simulink model "Trigger_FOC_Deadtime"  (R2022b)
settings: Solver=VariableStepAuto  StartTime=0.0  StopTime=0.5  RelTol=1e-3
PreLoadFcn:
  | % 沉沙motor:https://www.zhihu.com/people/gun-ne-ni
InitFcn:
  | %沉沙motor:https://www.zhihu.com/people/gun-ne-ni
  | 
  | deadtime = 2e-6;
undefined symbols (not defined in the file): Udc
libraries: spsGroundLib x1, spsPermanentMagnetSynchronousMachineLib x1, spsUniversalBridgeLib x1, spsDCVoltageSourceLib x1, sps_lib x1
settings Model: Creator=CSMotor  LastModifiedBy=CSMotor
settings DataIOCC: ReturnWorkspaceOutputs=off

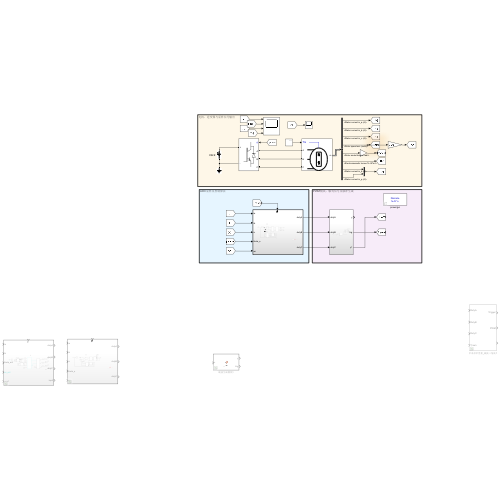
[thumbnail: Simulink's stored preview of the top-level diagram]
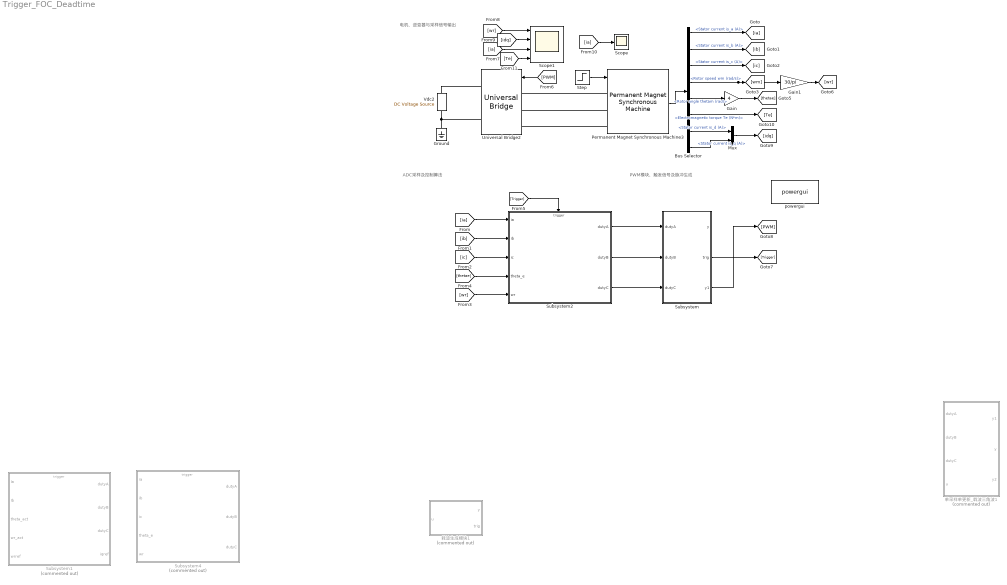
== system Trigger_FOC_Deadtime ==
  note: ADC采样及控制算法
  note: 电机、逆变器与采样信号输出
  note: PWM模块、触发信号及脉冲生成
  Bus Selector : BusSelector  OutputSignals=Stator current is_a (A),Stator current is_b (A),Stator current is_c (A),Rotor speed wm (rad/s),Rotor angle thetam (rad),Electromagnetic torque Te (N*m),Stator current is_d (A),Stator current is_q (A)
  Gain : Gain  Gain=4
  Gain1 : Gain  Gain=30/pi
  Ground : spsGroundLib/Ground  LConnTagsString=a
  Mux : Mux  Inputs=2
  Permanent Magnet Synchronous Machine3 : spsPermanentMagnetSynchronousMachineLib/Permanent Magnet Synchronous Machine  Description=沉沙motor:https://www.zhihu.com/people/gun-ne-ni  NbPhases=3  FluxDistribution=Sinusoidal  RotorType=Salient-pole  MechanicalLoad=Torque Tm  PresetModel="05:  8 Nm 300 Vdc 2000 RPM - 10 Nm"  ShowDetailedParameters=on  MeasurementBus=off  Resistance=0.9585  Inductance=8.5e-3  dqInductances=[0.004987 0.005513]  La=0.000835  MachineConstant=Flux linkage established by magnets (V.s)  Flux=0.1827  VoltageCst=132.5525  TorqueCst=1.0962  Flat=120  Mechanical=[0.0006329 0.0003035 4 0]  PolePairs=4  InitialConditions=[0,0, 0,0]  InitialConditions5ph=[0 0 0 0 0 0]  RefAngle=Aligned with phase A axis (original Park)  IterativeDiscreteModel=Trapezoidal non iterative  TsBlock=-1  TsPowergui=0
  Scope : Scope
  Scope1 : Scope  NumInputPorts=4
  Step : Step  Time=0.25  After=5  SampleTime=0
  Subsystem : Subsystem
  Subsystem1 : Subsystem  Commented=on
  Subsystem2 : Subsystem
  Subsystem4 : Subsystem  Commented=on
  Universal Bridge2 : spsUniversalBridgeLib/Universal Bridge  Description=沉沙motor:https://www.zhihu.com/people/gun-ne-ni  Arms=3  SnubberResistance=1e5  SnubberCapacitance=inf  Device=IGBT / Diodes  Ron=1e-3  Lon=0  ForwardVoltages="[  0  0  ]"  ForwardVoltage=0  GTOparameters=[ 10e-6 , 20e-6 ]  IGBTparameters=[ 1e-6 , 2e-6 ]  Measurements=None  Measurements_2=None  converterType=Rectifier
  Vdc2 : spsDCVoltageSourceLib/DC Voltage Source  Amplitude=300  Measurements=None
  powergui : sps_lib/powergui  Priority=1  SimulationMode=Discrete  SampleTime=1e-7  frequency=60  Iterations=50  frequencyindice=0  Pbase=100e6  ErrMax=1e-4  UnitsV=kV  UnitsW=MW  buscounter=0  FunctionMessages=off  echomessages=off  EnableUseOfTLC=off  CurrentSourceSwitches=off  DisableSnubberDevices=off  DisableRonSwitches=off  DisableVfSwitches=off  DisplayEquations=off  AutomaticDiscreteSolvers=off  SolverType=Tustin/Backward Euler (TBE)  Interpol=off  ExternalGateDelay=off  methode=off  Ts=100  x0status=blocks  SPID=on  SwTol=0  HookPort=off  NonlinearTolerance=1e-4  nMaxIteration=100  ContinueOnMaxIteration=off  RestoreLinks=warning  ResistiveCurrentMeasurement=off  Frange=[0:2:500]  Ylog=off  Xlog=on  ShowGrid=off  save=off  variable=ZData  structure=0  ZoomFFT=off  StartTime=0.0  cycles=1  DisplayStyle=1  fundamental=60  FreqAxis=off  MaxFrequency=1000  frequencyindicesteady=1  RmsSteady=1  display=off
  单采样单更新_载波三角波1 : Subsystem  Commented=on
      mask Display:
      | port_label('output',1,'Trigger')
      | port_label('output',2,'PWM')
      | 
      | 
      | 
      | port_label('input',1,'DutyA')
      | port_label('input',2,'DutyB')
      | port_label('input',3,'DutyC')
      | port_label('input',4,'Tpwm')
  载波生成模块1 : MATLAB Function  Commented=on  TreatAsAtomicUnit=on
  wires:
  Permanent Magnet Synchronous Machine3/1 -> Bus Selector/1
  Bus Selector/1 -> [ia]  "<Stator current is_a (A)>"
  Bus Selector/2 -> [ib]  "<Stator current is_b (A)>"
  Bus Selector/3 -> [ic]  "<Stator current is_c (A)>"
  Bus Selector/4 -> Gain1/1, [wm]  "<Rotor speed wm (rad/s)>"
  Bus Selector/5 -> Gain/1  "<Rotor angle thetam (rad)>"
  Gain/1 -> [thetae]
  Gain1/1 -> [wr]
  [PWM] -> Universal Bridge2/1
  [wr] -> Subsystem2/5(wr)
  [Trigger] -> Subsystem2/Trigger
  [ia] -> Subsystem2/1(ia)
  [ib] -> Subsystem2/2(ib)
  [ic] -> Subsystem2/3(ic)
  [thetae] -> Subsystem2/4(theta_e)
  Subsystem/2(trig) -> [Trigger]
  Subsystem2/1(dutyA) -> Subsystem/1(dutyA)
  Subsystem2/2(dutyB) -> Subsystem/2(dutyB)
  Subsystem2/3(dutyC) -> Subsystem/3(dutyC)
  Step/1 -> Permanent Magnet Synchronous Machine3/1
  [wr] -> Scope1/1
  [ia] -> Scope1/3
  Bus Selector/7 -> Mux/1  "<Stator current is_d (A)>"
  Bus Selector/8 -> Mux/2  "<Stator current is_q (A)>"
  Mux/1 -> [idq]
  [idq] -> Scope1/2
  Bus Selector/6 -> [Te]  "<Electromagnetic torque Te (N*m)>"
  [Te] -> Scope1/4
  [ia] -> Scope/1
  Subsystem/3(y1) -> [PWM]
  connections:
  Permanent Magnet Synchronous Machine3/LConn1 -- Universal Bridge2/LConn1
  Permanent Magnet Synchronous Machine3/LConn2 -- Universal Bridge2/LConn2
  Permanent Magnet Synchronous Machine3/LConn3 -- Universal Bridge2/LConn3
  Vdc2/RConn1 -- Universal Bridge2/RConn1
  Vdc2/LConn1 -- Ground/LConn1 -- Universal Bridge2/RConn2

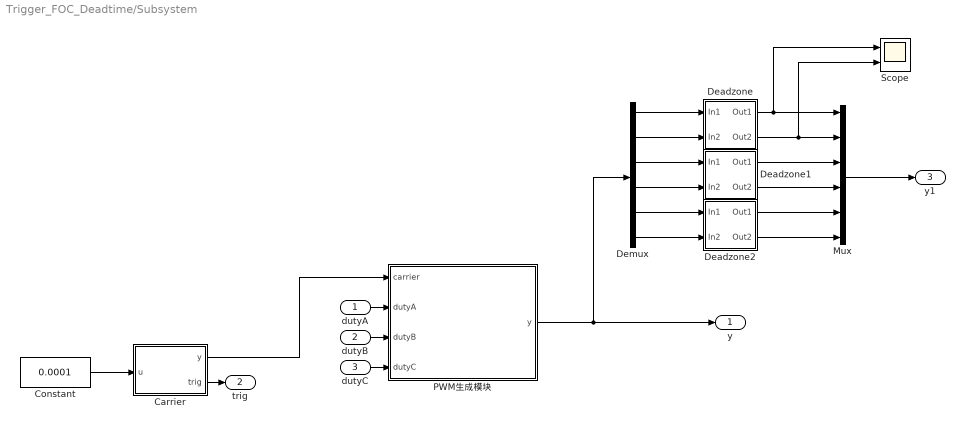
== system Trigger_FOC_Deadtime/Subsystem ==
  dutyA : Inport
  dutyB : Inport  Port=2
  dutyC : Inport  Port=3
  Carrier : MATLAB Function  Description=沉沙motor:https://www.zhihu.com/people/gun-ne-ni  TreatAsAtomicUnit=on
  Constant : Constant  Value=0.0001
  Deadzone : Subsystem
  Deadzone1 : Subsystem
  Deadzone2 : Subsystem
  Demux : Demux  Outputs=6
  Mux : Mux  Inputs=6
  PWM生成模块 : MATLAB Function  Description=沉沙motor:https://www.zhihu.com/people/gun-ne-ni  TreatAsAtomicUnit=on
  Scope : Scope  NumInputPorts=2
  y : Outport
  trig : Outport  Port=2
  y1 : Outport  Port=3
  wires:
  Carrier/1(y) -> PWM生成模块/1(carrier)
  PWM生成模块/1(y) -> Demux/1, y/1
  dutyC/1 -> PWM生成模块/4(dutyC)
  Constant/1 -> Carrier/1(u)
  dutyA/1 -> PWM生成模块/2(dutyA)
  dutyB/1 -> PWM生成模块/3(dutyB)
  Carrier/2(trig) -> trig/1
  Demux/1 -> Deadzone/1(In1)
  Demux/2 -> Deadzone/2(In2)
  Deadzone/2(Out2) -> Scope/2, Mux/2
  Deadzone/1(Out1) -> Scope/1, Mux/1
  Demux/3 -> Deadzone1/1(In1)
  Demux/4 -> Deadzone1/2(In2)
  Deadzone1/1(Out1) -> Mux/3
  Deadzone1/2(Out2) -> Mux/4
  Demux/5 -> Deadzone2/1(In1)
  Demux/6 -> Deadzone2/2(In2)
  Deadzone2/1(Out1) -> Mux/5
  Deadzone2/2(Out2) -> Mux/6
  Mux/1 -> y1/1

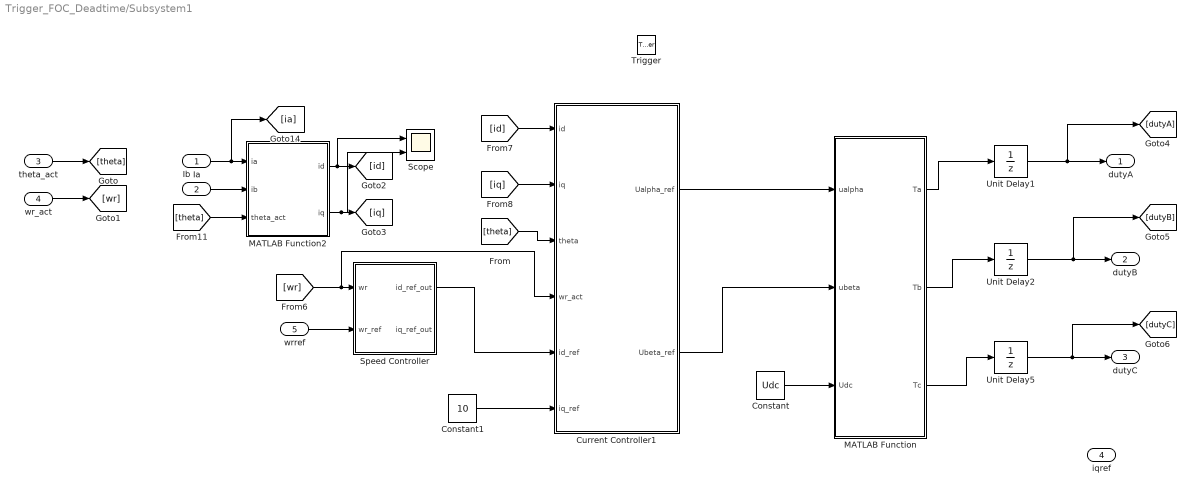
== system Trigger_FOC_Deadtime/Subsystem1 ==
  Ia : Inport
  Ib : Inport  Port=2
  theta_act : Inport  Port=3
  wr_act : Inport  Port=4
  wrref : Inport  Port=5
  Trigger : TriggerPort  VariantControl=(inherit)  PortDimensions=1
  Constant : Constant  Value=Udc
  Constant1 : Constant  Value=10
  Current Controller1 : MATLAB Function  TreatAsAtomicUnit=on
  MATLAB Function : MATLAB Function  TreatAsAtomicUnit=on
  MATLAB Function2 : MATLAB Function  TreatAsAtomicUnit=on
  Scope : Scope  NumInputPorts=2
  Speed Controller : MATLAB Function  TreatAsAtomicUnit=on
  Unit Delay1 : UnitDelay  InitialCondition=1e-4  SampleTime=-1  HasFrameUpgradeWarning=on
  Unit Delay2 : UnitDelay  InitialCondition=1e-4  SampleTime=-1  HasFrameUpgradeWarning=on
  Unit Delay5 : UnitDelay  InitialCondition=1e-4  SampleTime=-1  HasFrameUpgradeWarning=on
  dutyA : Outport
  dutyB : Outport  Port=2
  dutyC : Outport  Port=3
  iqref : Outport  Port=4
  wires:
  Constant1/1 -> Current Controller1/6(iq_ref)
  [iq] -> Current Controller1/2(iq)
  MATLAB Function2/1(id) -> [id], Scope/1
  MATLAB Function/2(Tb) -> Unit Delay2/1
  [id] -> Current Controller1/1(id)
  Unit Delay5/1 -> [dutyC], dutyC/1
  MATLAB Function/3(Tc) -> Unit Delay5/1
  Unit Delay1/1 -> [dutyA], dutyA/1
  Current Controller1/2(Ubeta_ref) -> MATLAB Function/2(ubeta)
  MATLAB Function/1(Ta) -> Unit Delay1/1
  MATLAB Function2/2(iq) -> [iq], Scope/2
  Ib/1 -> MATLAB Function2/2(ib)
  wrref/1 -> Speed Controller/2(wr_ref)
  Ia/1 -> [ia], MATLAB Function2/1(ia)
  [theta] -> MATLAB Function2/3(theta_act)
  [wr] -> Current Controller1/4(wr_act), Speed Controller/1(wr)
  Unit Delay2/1 -> [dutyB], dutyB/1
  [theta] -> Current Controller1/3(theta)
  Constant/1 -> MATLAB Function/3(Udc)
  Current Controller1/1(Ualpha_ref) -> MATLAB Function/1(ualpha)
  theta_act/1 -> [theta]
  Speed Controller/1(id_ref_out) -> Current Controller1/5(id_ref)
  wr_act/1 -> [wr]

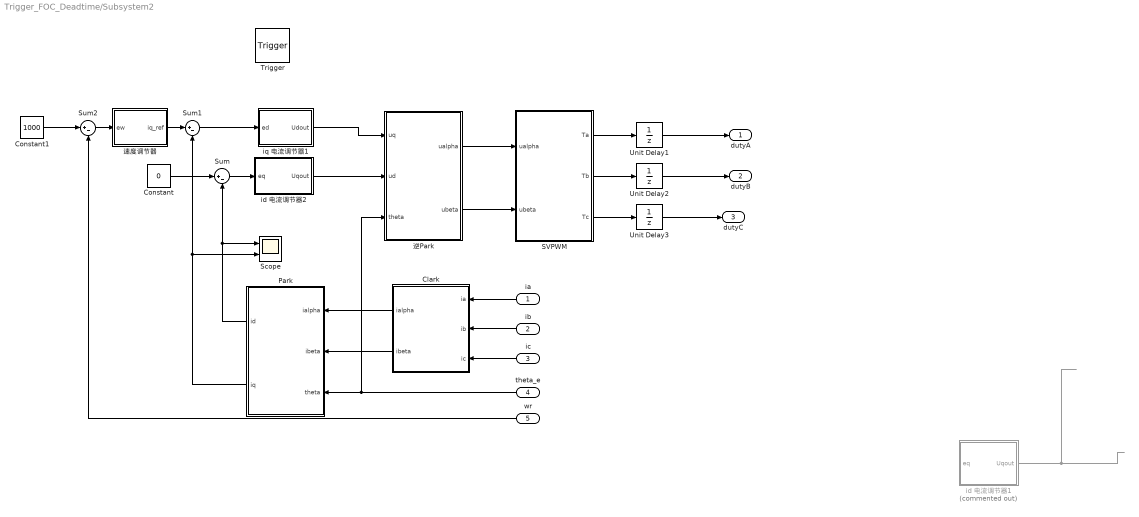
== system Trigger_FOC_Deadtime/Subsystem2 ==
  ia : Inport
  ib : Inport  Port=2
  ic : Inport  Port=3
  theta_e : Inport  Port=4
  wr : Inport  Port=5
  Trigger : TriggerPort  VariantControl=(inherit)  PortDimensions=1
  Clark : MATLAB Function  Description=沉沙motor:https://www.zhihu.com/people/gun-ne-ni  TreatAsAtomicUnit=on
  Constant : Constant  Value=0
  Constant1 : Constant  Value=1000
  Park : MATLAB Function  Description=沉沙motor:https://www.zhihu.com/people/gun-ne-ni  TreatAsAtomicUnit=on
  SVPWM : MATLAB Function  Description=沉沙motor:https://www.zhihu.com/people/gun-ne-ni  TreatAsAtomicUnit=on
  Scope : Scope  NumInputPorts=2
  Sum : Sum  Inputs=|+-
  Sum1 : Sum  Inputs=|+-
  Sum2 : Sum  Inputs=|+-
  Unit Delay1 : UnitDelay  InitialCondition=1e-4  SampleTime=-1  HasFrameUpgradeWarning=on
  Unit Delay2 : UnitDelay  InitialCondition=1e-4  SampleTime=-1  HasFrameUpgradeWarning=on
  Unit Delay3 : UnitDelay  InitialCondition=1e-4  SampleTime=-1  HasFrameUpgradeWarning=on
  id 电流调节器1 : MATLAB Function  Commented=on  TreatAsAtomicUnit=on
  id 电流调节器2 : MATLAB Function  Tag=s  Description=沉沙motor:https://www.zhihu.com/people/gun-ne-ni  TreatAsAtomicUnit=on
  iq 电流调节器1 : MATLAB Function  Description=沉沙motor:https://www.zhihu.com/people/gun-ne-ni  TreatAsAtomicUnit=on
  逆Park : MATLAB Function  Description=沉沙motor:https://www.zhihu.com/people/gun-ne-ni  TreatAsAtomicUnit=on
  速度调节器 : MATLAB Function  TreatAsAtomicUnit=on
  dutyA : Outport
  dutyB : Outport  Port=2
  dutyC : Outport  Port=3
  wires:
  id 电流调节器1/1(Uqout) -> ?
  SVPWM/3(Tc) -> Unit Delay3/1
  SVPWM/2(Tb) -> Unit Delay2/1
  SVPWM/1(Ta) -> Unit Delay1/1
  Constant1/1 -> Sum2/1
  wr/1 -> Sum2/2
  Sum2/1 -> 速度调节器/1(ew)
  Park/2(iq) -> Scope/2, Sum1/2
  Clark/2(ibeta) -> Park/2(ibeta)
  Clark/1(ialpha) -> Park/1(ialpha)
  theta_e/1 -> Park/3(theta), 逆Park/3(theta)
  ic/1 -> Clark/3(ic)
  ib/1 -> Clark/2(ib)
  ia/1 -> Clark/1(ia)
  逆Park/1(ualpha) -> SVPWM/1(ualpha)
  逆Park/2(ubeta) -> SVPWM/2(ubeta)
  Sum/1 -> id 电流调节器2/1(eq)
  Constant/1 -> Sum/1
  速度调节器/1(iq_ref) -> Sum1/1
  Sum1/1 -> iq 电流调节器1/1(ed)
  iq 电流调节器1/1(Udout) -> 逆Park/1(uq)
  id 电流调节器2/1(Uqout) -> 逆Park/2(ud)
  Park/1(id) -> Sum/2, Scope/1
  Unit Delay1/1 -> dutyA/1
  Unit Delay2/1 -> dutyB/1
  Unit Delay3/1 -> dutyC/1

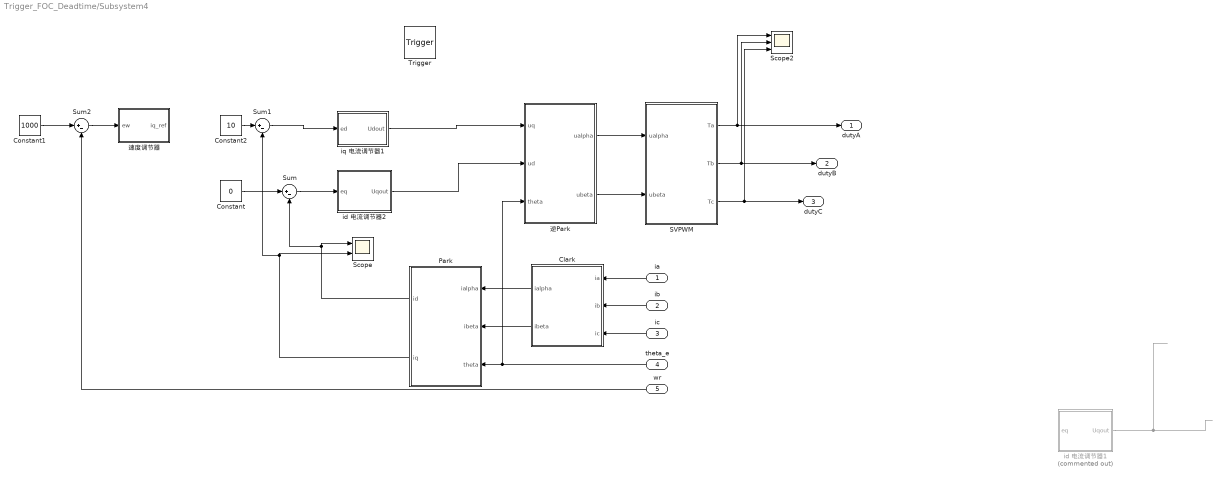
== system Trigger_FOC_Deadtime/Subsystem4 ==
  ia : Inport
  ib : Inport  Port=2
  ic : Inport  Port=3
  theta_e : Inport  Port=4
  wr : Inport  Port=5
  Trigger : TriggerPort  VariantControl=(inherit)  PortDimensions=1
  Clark : MATLAB Function  TreatAsAtomicUnit=on
  Constant : Constant  Value=0
  Constant1 : Constant  Value=1000
  Constant2 : Constant  Value=10
  Park : MATLAB Function  TreatAsAtomicUnit=on
  SVPWM : MATLAB Function  TreatAsAtomicUnit=on
  Scope : Scope  NumInputPorts=2
  Scope2 : Scope  NumInputPorts=3
  Sum : Sum  Inputs=|+-
  Sum1 : Sum  Inputs=|+-
  Sum2 : Sum  Inputs=|+-
  id 电流调节器1 : MATLAB Function  Commented=on  TreatAsAtomicUnit=on
  id 电流调节器2 : MATLAB Function  TreatAsAtomicUnit=on
  iq 电流调节器1 : MATLAB Function  TreatAsAtomicUnit=on
  逆Park : MATLAB Function  TreatAsAtomicUnit=on
  速度调节器 : MATLAB Function  TreatAsAtomicUnit=on
  dutyA : Outport
  dutyB : Outport  Port=2
  dutyC : Outport  Port=3
  wires:
  id 电流调节器2/1(Uqout) -> 逆Park/2(ud)
  iq 电流调节器1/1(Udout) -> 逆Park/1(uq)
  Sum1/1 -> iq 电流调节器1/1(ed)
  Constant2/1 -> Sum1/1
  Park/1(id) -> Scope/1, Sum/2
  Constant/1 -> Sum/1
  Sum/1 -> id 电流调节器2/1(eq)
  逆Park/2(ubeta) -> SVPWM/2(ubeta)
  逆Park/1(ualpha) -> SVPWM/1(ualpha)
  ia/1 -> Clark/1(ia)
  ib/1 -> Clark/2(ib)
  ic/1 -> Clark/3(ic)
  theta_e/1 -> 逆Park/3(theta), Park/3(theta)
  Clark/1(ialpha) -> Park/1(ialpha)
  Clark/2(ibeta) -> Park/2(ibeta)
  Park/2(iq) -> Scope/2, Sum1/2
  Sum2/1 -> 速度调节器/1(ew)
  wr/1 -> Sum2/2
  Constant1/1 -> Sum2/1
  SVPWM/1(Ta) -> Scope2/1, dutyA/1
  SVPWM/2(Tb) -> Scope2/2, dutyB/1
  SVPWM/3(Tc) -> Scope2/3, dutyC/1
  id 电流调节器1/1(Uqout) -> ?

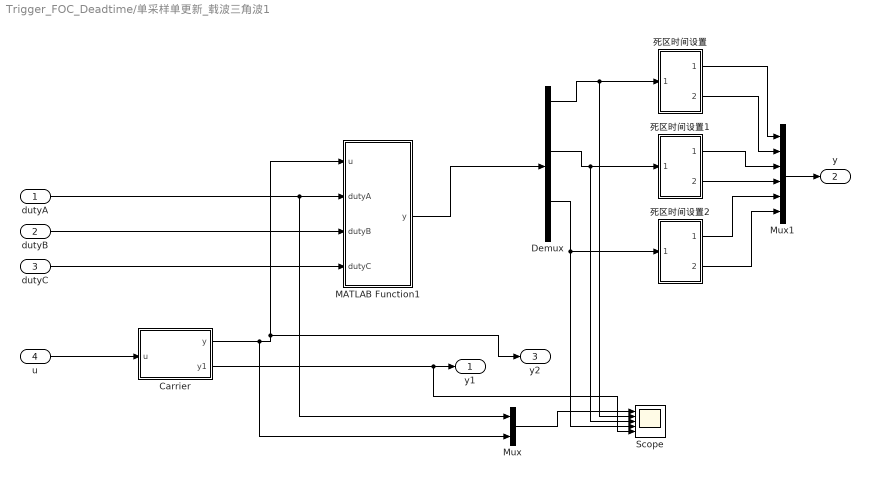
== system Trigger_FOC_Deadtime/单采样单更新_载波三角波1 ==
  dutyA : Inport
  dutyB : Inport  Port=2
  dutyC : Inport  Port=3
  u : Inport  Port=4
  Carrier : MATLAB Function  TreatAsAtomicUnit=on
  Demux : Demux  Outputs=6
  MATLAB Function1 : MATLAB Function  TreatAsAtomicUnit=on
  Mux : Mux  Inputs=2
  Mux1 : Mux  Inputs=6
  Scope : Scope  NumInputPorts=5
  死区时间设置 : Subsystem
  死区时间设置1 : Subsystem
  死区时间设置2 : Subsystem
  y1 : Outport
  y : Outport  Port=2
  y2 : Outport  Port=3
  wires:
  Carrier/2(y1) -> y1/1, Scope/5
  死区时间设置2/2(Out2) -> Mux1/6
  死区时间设置2/1(Out1) -> Mux1/5
  死区时间设置1/2(Out2) -> Mux1/4
  死区时间设置1/1(Out1) -> Mux1/3
  死区时间设置/2(Out2) -> Mux1/2
  死区时间设置/1(Out1) -> Mux1/1
  Demux/5 -> Scope/4, 死区时间设置2/1(In1)
  Demux/3 -> Scope/3, 死区时间设置1/1(In1)
  dutyA/1 -> Mux/1, MATLAB Function1/2(dutyA)
  MATLAB Function1/1(y) -> Demux/1
  u/1 -> Carrier/1(u)
  Carrier/1(y) -> Mux/2, y2/1, MATLAB Function1/1(u)
  dutyB/1 -> MATLAB Function1/3(dutyB)
  dutyC/1 -> MATLAB Function1/4(dutyC)
  Demux/1 -> Scope/2, 死区时间设置/1(In1)
  Mux/1 -> Scope/1
  Mux1/1 -> y/1

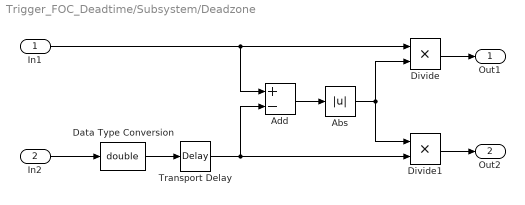
== system Trigger_FOC_Deadtime/Subsystem/Deadzone ==
  In1 : Inport
  In2 : Inport  Port=2
  Abs : Abs  SaturateOnIntegerOverflow=off
  Add : Sum  Inputs=+-
  Data Type Conversion : DataTypeConversion  OutDataTypeStr=double  SaturateOnIntegerOverflow=off  RndMeth=Floor
  Divide : Product  Inputs=**
  Divide1 : Product  Inputs=**
  Transport Delay : TransportDelay  DelayTime=2e-6
  Out1 : Outport  VectorParamsAs1DForOutWhenUnconnected=off
  Out2 : Outport  Port=2  VectorParamsAs1DForOutWhenUnconnected=off
  wires:
  Abs/1 -> Divide1/1, Divide/2
  Data Type Conversion/1 -> Transport Delay/1
  Add/1 -> Abs/1
  Transport Delay/1 -> Add/2, Divide1/2
  Divide/1 -> Out1/1
  In2/1 -> Data Type Conversion/1
  In1/1 -> Divide/1, Add/1
  Divide1/1 -> Out2/1

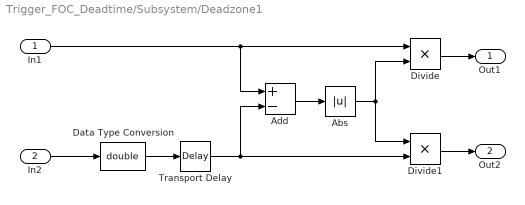
== system Trigger_FOC_Deadtime/Subsystem/Deadzone1 ==
  In1 : Inport
  In2 : Inport  Port=2
  Abs : Abs  SaturateOnIntegerOverflow=off
  Add : Sum  Inputs=+-
  Data Type Conversion : DataTypeConversion  OutDataTypeStr=double  SaturateOnIntegerOverflow=off  RndMeth=Floor
  Divide : Product  Inputs=**
  Divide1 : Product  Inputs=**
  Transport Delay : TransportDelay  DelayTime=2e-6
  Out1 : Outport  VectorParamsAs1DForOutWhenUnconnected=off
  Out2 : Outport  Port=2  VectorParamsAs1DForOutWhenUnconnected=off
  wires:
  Divide1/1 -> Out2/1
  In1/1 -> Add/1, Divide/1
  In2/1 -> Data Type Conversion/1
  Divide/1 -> Out1/1
  Transport Delay/1 -> Divide1/2, Add/2
  Add/1 -> Abs/1
  Data Type Conversion/1 -> Transport Delay/1
  Abs/1 -> Divide/2, Divide1/1

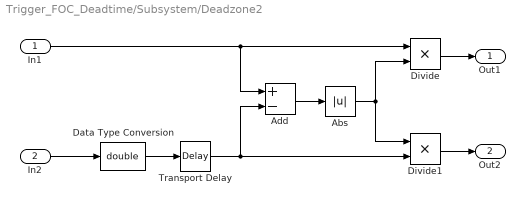
== system Trigger_FOC_Deadtime/Subsystem/Deadzone2 ==
  In1 : Inport
  In2 : Inport  Port=2
  Abs : Abs  SaturateOnIntegerOverflow=off
  Add : Sum  Inputs=+-
  Data Type Conversion : DataTypeConversion  OutDataTypeStr=double  SaturateOnIntegerOverflow=off  RndMeth=Floor
  Divide : Product  Inputs=**
  Divide1 : Product  Inputs=**
  Transport Delay : TransportDelay  DelayTime=2e-6
  Out1 : Outport  VectorParamsAs1DForOutWhenUnconnected=off
  Out2 : Outport  Port=2  VectorParamsAs1DForOutWhenUnconnected=off
  wires:
  Abs/1 -> Divide1/1, Divide/2
  Data Type Conversion/1 -> Transport Delay/1
  Add/1 -> Abs/1
  Transport Delay/1 -> Add/2, Divide1/2
  Divide/1 -> Out1/1
  In2/1 -> Data Type Conversion/1
  In1/1 -> Divide/1, Add/1
  Divide1/1 -> Out2/1

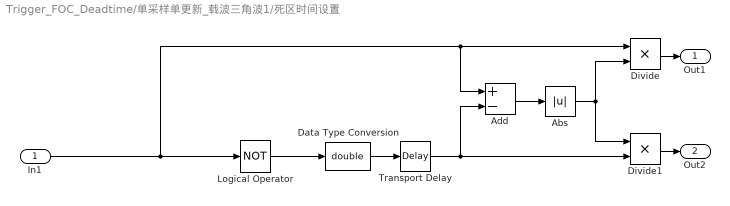
== system Trigger_FOC_Deadtime/单采样单更新_载波三角波1/死区时间设置 ==
  In1 : Inport
  Abs : Abs  SaturateOnIntegerOverflow=off
  Add : Sum  Inputs=+-
  Data Type Conversion : DataTypeConversion  OutDataTypeStr=double  SaturateOnIntegerOverflow=off  RndMeth=Floor
  Divide : Product  Inputs=**
  Divide1 : Product  Inputs=**
  Logical Operator : Logic  Operator=NOT  AllPortsSameDT=off  OutDataTypeStr=boolean
  Transport Delay : TransportDelay  DelayTime=deadtime
  Out1 : Outport  VectorParamsAs1DForOutWhenUnconnected=off
  Out2 : Outport  Port=2  VectorParamsAs1DForOutWhenUnconnected=off
  wires:
  Add/1 -> Abs/1
  Divide1/1 -> Out2/1
  Logical Operator/1 -> Data Type Conversion/1
  Divide/1 -> Out1/1
  Abs/1 -> Divide/2, Divide1/1
  In1/1 -> Add/1, Divide/1, Logical Operator/1
  Transport Delay/1 -> Divide1/2, Add/2
  Data Type Conversion/1 -> Transport Delay/1

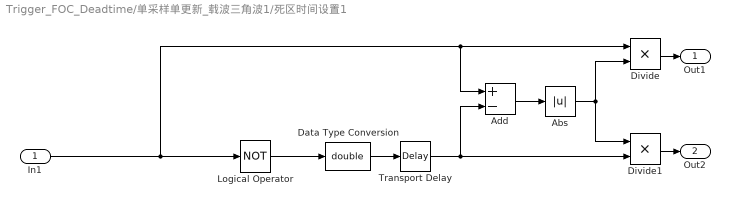
== system Trigger_FOC_Deadtime/单采样单更新_载波三角波1/死区时间设置1 ==
  In1 : Inport
  Abs : Abs  SaturateOnIntegerOverflow=off
  Add : Sum  Inputs=+-
  Data Type Conversion : DataTypeConversion  OutDataTypeStr=double  SaturateOnIntegerOverflow=off  RndMeth=Floor
  Divide : Product  Inputs=**
  Divide1 : Product  Inputs=**
  Logical Operator : Logic  Operator=NOT  AllPortsSameDT=off  OutDataTypeStr=boolean
  Transport Delay : TransportDelay  DelayTime=deadtime
  Out1 : Outport  VectorParamsAs1DForOutWhenUnconnected=off
  Out2 : Outport  Port=2  VectorParamsAs1DForOutWhenUnconnected=off
  wires:
  Data Type Conversion/1 -> Transport Delay/1
  Transport Delay/1 -> Add/2, Divide1/2
  In1/1 -> Logical Operator/1, Divide/1, Add/1
  Abs/1 -> Divide1/1, Divide/2
  Divide/1 -> Out1/1
  Logical Operator/1 -> Data Type Conversion/1
  Divide1/1 -> Out2/1
  Add/1 -> Abs/1

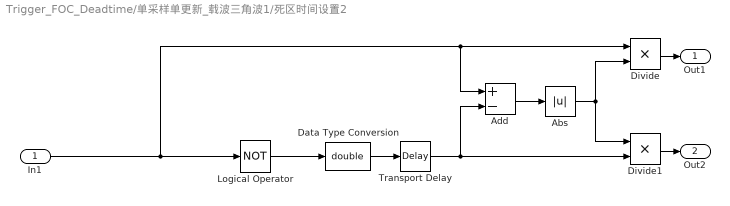
== system Trigger_FOC_Deadtime/单采样单更新_载波三角波1/死区时间设置2 ==
  In1 : Inport
  Abs : Abs  SaturateOnIntegerOverflow=off
  Add : Sum  Inputs=+-
  Data Type Conversion : DataTypeConversion  OutDataTypeStr=double  SaturateOnIntegerOverflow=off  RndMeth=Floor
  Divide : Product  Inputs=**
  Divide1 : Product  Inputs=**
  Logical Operator : Logic  Operator=NOT  AllPortsSameDT=off  OutDataTypeStr=boolean
  Transport Delay : TransportDelay  DelayTime=deadtime
  Out1 : Outport  VectorParamsAs1DForOutWhenUnconnected=off
  Out2 : Outport  Port=2  VectorParamsAs1DForOutWhenUnconnected=off
  wires:
  Add/1 -> Abs/1
  Divide1/1 -> Out2/1
  Logical Operator/1 -> Data Type Conversion/1
  Divide/1 -> Out1/1
  Abs/1 -> Divide/2, Divide1/1
  In1/1 -> Add/1, Divide/1, Logical Operator/1
  Transport Delay/1 -> Divide1/2, Add/2
  Data Type Conversion/1 -> Transport Delay/1

== matlab function Trigger_FOC_Deadtime/Subsystem4/Park ==
  data: ialpha input; id output; ibeta input; theta input; iq output
function [id, iq] = fcn(ialpha, ibeta, theta)
%#codegen
id =  ialpha*cos(theta) + ibeta*sin(theta);
iq = -ialpha*sin(theta) + ibeta*cos(theta);

== matlab function Trigger_FOC_Deadtime/Subsystem2/Clark ==
  data: ia input; ialpha output; ib input; ic input; ibeta output
function [ialpha, ibeta] = fcn_clarke(ia, ib, ic)
%#codegen
ialpha = (2/3) * (ia - 0.5*ib - 0.5*ic);
ibeta  = (2/3) * (sqrt(3)/2*ib - sqrt(3)/2*ic);

== matlab function Trigger_FOC_Deadtime/Subsystem/PWM生成模块 ==
  data: carrier input; y output; dutyA input; dutyB input; dutyC input
function y = fcn(carrier, dutyA, dutyB, dutyC)
%#codegen
ref  = carrier;
CMPA = dutyA;
CMPB = dutyB;
CMPC = dutyC;

Ta1 = 0;  Ta2 = 0;
Tb1 = 0;  Tb2 = 0;
Tc1 = 0;  Tc2 = 0;

if ref <= CMPA
    Ta1 = 1;  Ta2 = 0;
else
    Ta1 = 0;  Ta2 = 1;
end

if ref <= CMPB
    Tb1 = 1;  Tb2 = 0;
else
    Tb1 = 0;  Tb2 = 1;
end

if ref <= CMPC
    Tc1 = 1;  Tc2 = 0;
else
    Tc1 = 0;  Tc2 = 1;
end

y = [Ta1; Ta2; Tb1; Tb2; Tc1; Tc2];

== matlab function Trigger_FOC_Deadtime/Subsystem/Carrier ==
  data: u input; y output; trig output
function [y, trig] = carrier(u)
%#codegen
persistent cnt dir
if isempty(cnt)
    cnt = 0;
    dir = 1;
end
Tdis = 1e-7;
n  = round(u/Tdis);
nh = n/2;

y = cnt/nh;
trig = (cnt == nh);

cnt = cnt + dir;
if cnt >= nh
    cnt = nh;
    dir = -1;
elseif cnt <= 0
    cnt = 0;
    dir = 1;
end

== matlab function Trigger_FOC_Deadtime/载波生成模块1 ==
  data: u input; y output; trig output
function [y, trig] = carrier(u)
%#codegen
persistent cnt dir
if isempty(cnt)
    cnt = 0;
    dir = 1;
end
Tdis = 1e-7;
n  = round(u/Tdis);
nh = n/2;

y = cnt/nh;
trig = (cnt == nh);

cnt = cnt + dir;
if cnt >= nh
    cnt = nh;
    dir = -1;
elseif cnt <= 0
    cnt = 0;
    dir = 1;
end

== matlab function Trigger_FOC_Deadtime/Subsystem1/Current Controller1 ==
  data: id input; iq input; theta input; wr_act input; id_ref input; iq_ref input; Ualpha_ref output; Ubeta_ref output
function [Ualpha_ref,Ubeta_ref]  = fcn(id, iq, theta, wr_act, id_ref, iq_ref)
    persistent int_d int_q Kp Ki Ld Lq Phif Pn Tsc U_max Rs
    if isempty(int_d)
        int_d = 0;
        int_q = 0;
        Ld = 0.08e-3;
        Lq = 0.08e-3;
        Rs = 0.06;
        Phif = 0.003749;
        Pn = 5;
        Tsc = 0.0001;
        U_max = 24/sqrt(3);
    end
    
        Kp = Ld/4/Tsc;
        Ki = Rs/3/Tsc;

    we = wr_act * (2*pi/60) * Pn;
    
    err_d = id_ref - id;
    err_q = iq_ref - iq;
    
    int_d = int_d + Ki * err_d * Tsc;
    int_q = int_q + Ki * err_q * Tsc;

    %%%%%%%%% 积分限幅 %%%%%%%%%%%%
    if int_d > U_max 
        int_d = U_max;
    elseif int_d < -U_max
        int_d = -U_max;
    else
    end

    if int_q > U_max 
        int_q = U_max;
    elseif int_q < -U_max
        int_q = -U_max;
    else
    end

    %%%%%%%%%%% PI 输出 %%%%%%%%%%%
    Ud_raw = Kp * err_d + int_d;
    Uq_raw = Kp * err_q + int_q;
    
    
    U_mag = sqrt(Ud_raw^2 + Uq_raw^2);
    if U_mag > U_max
        scale = U_max / U_mag;
        Udout = Ud_raw * scale;
        Uqout = Uq_raw * scale;
    else
        Udout = Ud_raw;
        Uqout = Uq_raw;
    end
    
    theta_comp = theta + 1.5 * we * Tsc;
    Ualpha_ref = Udout * cos(theta_comp) - Uqout * sin(theta_comp);
    Ubeta_ref  = Udout * sin(theta_comp) + Uqout * cos(theta_comp);
end

== matlab function Trigger_FOC_Deadtime/Subsystem4/SVPWM ==
  data: ualpha input; Ta output; ubeta input; Tb output; Tc output
function [Ta, Tb, Tc] = fcn_svpwm(ualpha, ubeta)
%#codegen
SQRT3     = 1.73205080757;
SQRT3_INV = 0.57735026919;
Udc  = 300;

volAlphaNorm = ualpha/Udc*SQRT3;
volBetaNorm  = ubeta /Udc*SQRT3;

voltU = volAlphaNorm;
voltV = -0.5*volAlphaNorm + SQRT3*0.5*volBetaNorm;
voltW = -0.5*volAlphaNorm - SQRT3*0.5*volBetaNorm;

voltMax = max([voltU, voltV, voltW]);
voltMin = min([voltU, voltV, voltW]);
voltZero = -0.5*(voltMax + voltMin);

dutyU = SQRT3_INV*(voltU + voltZero) + 0.5;
dutyV = SQRT3_INV*(voltV + voltZero) + 0.5;
dutyW = SQRT3_INV*(voltW + voltZero) + 0.5;

Ta = min(max(dutyU, 0), 1);
Tb = min(max(dutyV, 0), 1);
Tc = min(max(dutyW, 0), 1);

== matlab function Trigger_FOC_Deadtime/Subsystem4/id 电流调节器1 ==
  data: eq input; Uqout output
function Uqout = fcn_pi_q(eq)
%#codegen
Lq  = 0.005513;
Rs  = 0.9585;
Tsc = 0.0001;
Udc = 300;

Kpq = Lq/(3*Tsc);
Kiq = Rs/(3*Tsc);
Umax = max(Udc,0)/sqrt(3);

persistent int_q
if isempty(int_q)
    int_q = 0;
end

int_q = int_q + Kiq*eq*Tsc;

if int_q >  Umax, int_q =  Umax; end
if int_q < -Umax, int_q = -Umax; end

Uqout = Kpq*eq + int_q;

if Uqout >  Umax, Uqout =  Umax; end
if Uqout < -Umax, Uqout = -Umax; end

== matlab function Trigger_FOC_Deadtime/Subsystem1/MATLAB Function ==
  data: ualpha input; Ta output; ubeta input; Tb output; Tc output; Udc input
function [Ta, Tb, Tc] = fcn_svpwm(ualpha, ubeta, Udc)
%#codegen
SQRT3     = 1.73205080757;
SQRT3_INV = 0.57735026919;

volAlphaNorm = ualpha/Udc*SQRT3;
volBetaNorm  = ubeta/Udc*SQRT3;

voltU = volAlphaNorm;
voltV = -0.5*volAlphaNorm + SQRT3*0.5*volBetaNorm;
voltW = -0.5*volAlphaNorm - SQRT3*0.5*volBetaNorm;

voltMax = max([voltU, voltV, voltW]);
voltMin = min([voltU, voltV, voltW]);
voltZero = -0.5*(voltMax + voltMin);

dutyU = SQRT3_INV*(voltU + voltZero) + 0.5;
dutyV = SQRT3_INV*(voltV + voltZero) + 0.5;
dutyW = SQRT3_INV*(voltW + voltZero) + 0.5;

Ta = min(max(dutyU, 0), 1);
Tb = min(max(dutyV, 0), 1);
Tc = min(max(dutyW, 0), 1);

== matlab function Trigger_FOC_Deadtime/Subsystem2/Park ==
  data: ialpha input; id output; ibeta input; theta input; iq output
function [id, iq] = fcn(ialpha, ibeta, theta)
%#codegen
id =  ialpha*cos(theta) + ibeta*sin(theta);
iq = -ialpha*sin(theta) + ibeta*cos(theta);

== matlab function Trigger_FOC_Deadtime/Subsystem2/SVPWM ==
  data: ualpha input; Ta output; ubeta input; Tb output; Tc output
function [Ta, Tb, Tc] = fcn_svpwm(ualpha, ubeta)
%#codegen
SQRT3     = 1.73205080757;
SQRT3_INV = 0.57735026919;
Udc  = 300;

volAlphaNorm = ualpha/Udc*SQRT3;
volBetaNorm  = ubeta /Udc*SQRT3;

voltU = volAlphaNorm;
voltV = -0.5*volAlphaNorm + SQRT3*0.5*volBetaNorm;
voltW = -0.5*volAlphaNorm - SQRT3*0.5*volBetaNorm;

voltMax = max([voltU, voltV, voltW]);
voltMin = min([voltU, voltV, voltW]);
voltZero = -0.5*(voltMax + voltMin);

dutyU = SQRT3_INV*(voltU + voltZero) + 0.5;
dutyV = SQRT3_INV*(voltV + voltZero) + 0.5;
dutyW = SQRT3_INV*(voltW + voltZero) + 0.5;

Ta = min(max(dutyU, 0), 1);
Tb = min(max(dutyV, 0), 1);
Tc = min(max(dutyW, 0), 1);

== matlab function Trigger_FOC_Deadtime/Subsystem2/id 电流调节器1 ==
  data: eq input; Uqout output
function Uqout = fcn_pi_q(eq)
%#codegen
Lq  = 0.005513;
Rs  = 0.9585;
Tsc = 0.0001;
Udc = 300;

Kpq = Lq/(3*Tsc);
Kiq = Rs/(3*Tsc);
Umax = max(Udc,0)/sqrt(3);

persistent int_q
if isempty(int_q)
    int_q = 0;
end

int_q = int_q + Kiq*eq*Tsc;

if int_q >  Umax, int_q =  Umax; end
if int_q < -Umax, int_q = -Umax; end

Uqout = Kpq*eq + int_q;

if Uqout >  Umax, Uqout =  Umax; end
if Uqout < -Umax, Uqout = -Umax; end

== matlab function Trigger_FOC_Deadtime/Subsystem2/iq 电流调节器1 ==
  data: ed input; Udout output
function Udout = fcn_pi_d(ed)
%#codegen
Ld  = 0.004987;
Rs  = 0.9585;
Tsc = 0.0001;
Udc = 300;

Kpd = Ld/(3*Tsc);
Kid = Rs/(3*Tsc);
Umax = max(Udc,0)/sqrt(3);

persistent int_d
if isempty(int_d)
    int_d = 0;
end

int_d = int_d + Kid*ed*Tsc;

if int_d >  Umax, int_d =  Umax; end
if int_d < -Umax, int_d = -Umax; end

Udout = Kpd*ed + int_d;

if Udout >  Umax, Udout =  Umax; end
if Udout < -Umax, Udout = -Umax; end

== matlab function Trigger_FOC_Deadtime/Subsystem2/逆Park ==
  data: uq input; ud input; ualpha output; theta input; ubeta output
function [ualpha, ubeta] = fcn_invpark(uq, ud, theta)
%#codegen
ualpha = ud*cos(theta) - uq*sin(theta);
ubeta  = ud*sin(theta) + uq*cos(theta);

== matlab function Trigger_FOC_Deadtime/Subsystem2/速度调节器 ==
  data: ew input; iq_ref output
function iq_ref = fcn_w(ew)
%#codegen
Kp = 0.15;
Ki = 10;
Ts = 0.0001;

Imax    = 10;
int_lim = Imax/Ki;

persistent int_w
if isempty(int_w)
    int_w = 0;
end

int_w = int_w + ew*Ts;

if int_w >  int_lim, int_w =  int_lim; end
if int_w < -int_lim, int_w = -int_lim; end

iq_ref = Kp*ew + Ki*int_w;

if iq_ref >  Imax, iq_ref =  Imax; end
if iq_ref < -Imax, iq_ref = -Imax; end

== matlab function Trigger_FOC_Deadtime/Subsystem1/MATLAB Function2 ==
  data: ia input; ib input; theta_act input; id output; iq output
function[id,iq] = fcn(ia,ib,theta_act)
%%%%%%%%%%%%%%%%%%% theta 依据控制模式分流 %%%%%%%%%%%%%%%

    theta = theta_act;    

%%%%%%%%%%%%%%%%%%%%  clark + park %%%%%%%%%%%%%%%%%%%%%%%%%%%

ialpha = ia;                                         %3/2变换
ibeta = sqrt(3)/3*ia+2*sqrt(3)/3*ib;
id = ialpha * cos(theta)+ ibeta*sin(theta);          %帕克变换
iq = ialpha * -sin(theta)+ ibeta*cos(theta);

== matlab function Trigger_FOC_Deadtime/Subsystem1/Speed Controller ==
  data: wr input; id_ref_out output; iq_ref_out output; wr_ref input
function[id_ref_out,iq_ref_out] = fcn(wr,wr_ref)

persistent Kp_speed Ki_speed wr_inter_old Tsc 
if isempty(Kp_speed)
wr_inter_old = 0;  % 转速环PI积分回路储存值
Kp_speed =0.3;    % 转速环PI参数
Ki_speed =10;
Tsc = 0.0001;
end 
iq_limit = 11.5;

% %%%%%%%%%%%%%%%%%%%%  speed loop %%%%%%%%%%%%%%%%%%%%%%%%%%%%%%
erro_wr = wr_ref - wr ;                             %转速环PI调节器
wr_inter_old = wr_inter_old + Ki_speed*erro_wr*Tsc;
iq_ref = Kp_speed*erro_wr + wr_inter_old; 
if wr_inter_old>=iq_limit                           %% 积分限幅值
   wr_inter_old = iq_limit;
elseif wr_inter_old <=-iq_limit
    wr_inter_old  = -iq_limit;
end

if iq_ref>=iq_limit                                 %% 转速环限幅值
   iq_ref = iq_limit;
elseif iq_ref<=-iq_limit
    iq_ref = -iq_limit;
end
id_ref = 0;


iq_ref_out = iq_ref;
id_ref_out = id_ref;

== matlab function Trigger_FOC_Deadtime/Subsystem4/id 电流调节器2 ==
  data: eq input; Uqout output
function Uqout = fcn_pi_q(eq)
%#codegen
Lq  = 0.005513;
Rs  = 0.9585;
Tsc = 0.0001;
Udc = 300;

Kpq = Lq/(3*Tsc);
Kiq = Rs/(3*Tsc);
Umax = max(Udc,0)/sqrt(3);

persistent int_q
if isempty(int_q)
    int_q = 0;
end

int_q = int_q + Kiq*eq*Tsc;

if int_q >  Umax, int_q =  Umax; end
if int_q < -Umax, int_q = -Umax; end

Uqout = Kpq*eq + int_q;

if Uqout >  Umax, Uqout =  Umax; end
if Uqout < -Umax, Uqout = -Umax; end

== matlab function Trigger_FOC_Deadtime/Subsystem4/iq 电流调节器1 ==
  data: ed input; Udout output
function Udout = fcn_pi_d(ed)
%#codegen
Ld  = 0.004987;
Rs  = 0.9585;
Tsc = 0.0001;
Udc = 300;

Kpd = Ld/(3*Tsc);
Kid = Rs/(3*Tsc);
Umax = max(Udc,0)/sqrt(3);

persistent int_d
if isempty(int_d)
    int_d = 0;
end

int_d = int_d + Kid*ed*Tsc;

if int_d >  Umax, int_d =  Umax; end
if int_d < -Umax, int_d = -Umax; end

Udout = Kpd*ed + int_d;

if Udout >  Umax, Udout =  Umax; end
if Udout < -Umax, Udout = -Umax; end

== matlab function Trigger_FOC_Deadtime/Subsystem4/逆Park ==
  data: uq input; ud input; ualpha output; theta input; ubeta output
function [ualpha, ubeta] = fcn_invpark(uq, ud, theta)
%#codegen
ualpha = ud*cos(theta) - uq*sin(theta);
ubeta  = ud*sin(theta) + uq*cos(theta);

== matlab function Trigger_FOC_Deadtime/Subsystem4/速度调节器 ==
  data: ew input; iq_ref output
function iq_ref = fcn_w(ew)
%#codegen
Kp = 0.15;
Ki = 10;
Ts = 0.0001;

Imax    = 10;
int_lim = Imax/Ki;

persistent int_w
if isempty(int_w)
    int_w = 0;
end

int_w = int_w + ew*Ts;

if int_w >  int_lim, int_w =  int_lim; end
if int_w < -int_lim, int_w = -int_lim; end

iq_ref = Kp*ew + Ki*int_w;

if iq_ref >  Imax, iq_ref =  Imax; end
if iq_ref < -Imax, iq_ref = -Imax; end

== matlab function Trigger_FOC_Deadtime/单采样单更新_载波三角波1/Carrier ==
  data: u input; y output; y1 output; Ts parameter
function [y, y1] = carrier(u,Ts)
%#codegen

persistent  count clock
if isempty(count)
    count=0;
    clock = 0;
end

n=round(u/Ts);   % 累加步数
y1=0;
y=count/n*2;
clock = clock + 1;
if clock <= n/2
    count = count + 1;
else 
    count = count - 1;
    
end

if clock  <=1
    y1 = 0;
elseif clock <= (n/2+1) && clock> (n/2-1)
    y1 = 1;  % 此处设为1 即为顶点和低点都有触发信号；
else
    y1 = 0;
end

if clock>=n
    clock=0;  
end

== matlab function Trigger_FOC_Deadtime/单采样单更新_载波三角波1/MATLAB Function1 ==
  data: u input; y output; dutyA input; dutyB input; dutyC input
function y = fcn(u,dutyA,dutyB,dutyC)

ref = u;              % 载波
CMPA = 1-dutyA;
CMPB = 1-dutyB;
CMPC = 1-dutyC;
Ta1=0;
Ta2=0;
Tb1=0;
Tb2=0;
Tc1=0;
Tc2=0;
if ref>=CMPA            % ref 就是一个三角波发生器  A相PWM波形成  累加的过程中 Taon 大于了三角波  就 A相下桥臂通 上桥臂关
    Ta1=1;            % 此时对应的epwm模块的逻辑是，在上升过程中，当CMPA = TPRD时，置为1；在下降的过程中，当CMPA = TPRD时，置为0；
    Ta2=0;                   %所以输入的值越大实际占空比越小；
elseif ref<CMPA
    Ta1=0;
    Ta2=1;
end

if ref>=CMPB
    Tb1=1;
    Tb2=0;
elseif ref<CMPB
    Tb1=0;
    Tb2=1;
end

if ref>=CMPC
    Tc1=1;
    Tc2=0;
elseif ref<CMPC
    Tc1=0;
    Tc2=1;
end

y=[Ta1;Ta2;Tb1;Tb2;Tc1;Tc2];

== matlab function Trigger_FOC_Deadtime/Subsystem2/id 电流调节器2 ==
  data: eq input; Uqout output
function Uqout = fcn_pi_q(eq)
%#codegen
Lq  = 0.005513;
Rs  = 0.9585;
Tsc = 0.0001;
Udc = 300;

Kpq = Lq/(3*Tsc);
Kiq = Rs/(3*Tsc);
Umax = max(Udc,0)/sqrt(3);

persistent int_q
if isempty(int_q)
    int_q = 0;
end

int_q = int_q + Kiq*eq*Tsc;

if int_q >  Umax, int_q =  Umax; end
if int_q < -Umax, int_q = -Umax; end

Uqout = Kpq*eq + int_q;

if Uqout >  Umax, Uqout =  Umax; end
if Uqout < -Umax, Uqout = -Umax; end

== matlab function Trigger_FOC_Deadtime/Subsystem4/Clark ==
  data: ia input; ialpha output; ib input; ic input; ibeta output
function [ialpha, ibeta] = fcn_clarke(ia, ib, ic)
%#codegen
ialpha = (2/3) * (ia - 0.5*ib - 0.5*ic);
ibeta  = (2/3) * (sqrt(3)/2*ib - sqrt(3)/2*ic);
